simulink model "Oldham_Coupling"  (R2024b)
settings: Solver=ode15s  StartTime=0.0  StopTime=4  MaxStep=0.02  RelTol=1e-3
undefined symbols (not defined in the file or in its folder): X, Y, Z
libraries: sm_lib x14, nesl_utility x2, simulink x1
settings Model: Creator=admin  LastModifiedBy=admin

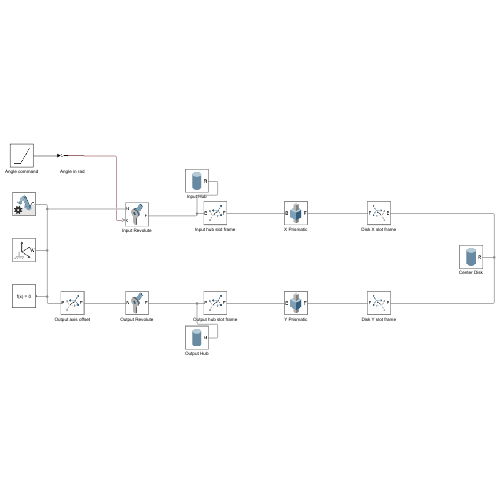
[thumbnail: Simulink's stored preview of the top-level diagram]
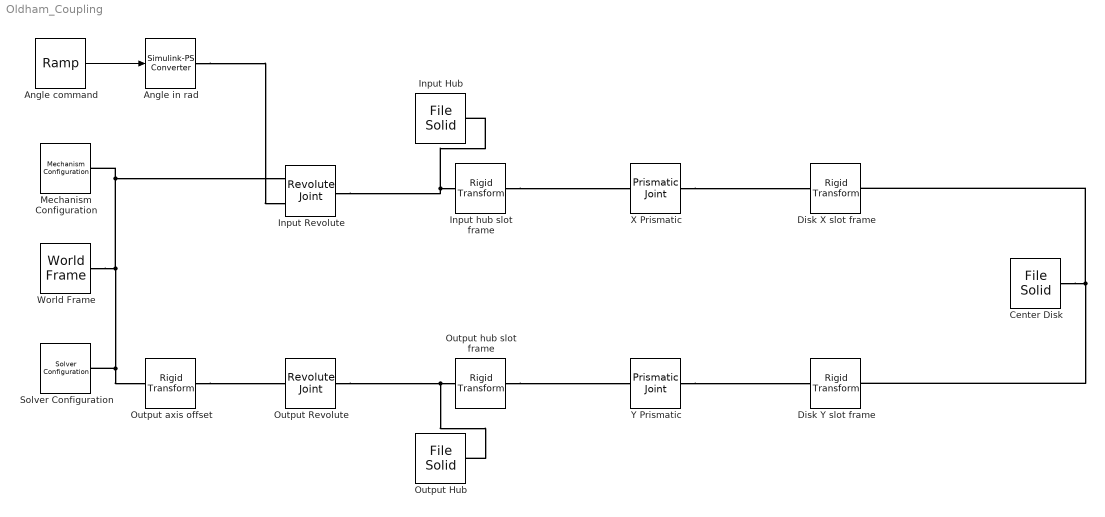
== system Oldham_Coupling ==
  Angle command : simulink/Sources/Ramp  slope=pi  start=0  InitialOutput=0
  Angle in rad : nesl_utility/Simulink-PS Converter  PhysicalDomain=network_engine_domain  SubClassName=ps_input  LeftPortType=input  RightPortType=output  PseudoPeriodic=off  Frequencies=[]  NoiseDistribution=none  NoiseParameters=[]  Unit=rad  AffineConversion=off  FilteringAndDerivatives=filter  SimscapeFilterOrder=2  InputFilterTimeConstant=0.001  UdotUserProvided=0
  Center Disk : sm_lib/Body Elements/File Solid  InertiaType=CalculateFromGeometry  BasedOnType=Density  Density=1000  DensityUnits=kg/m^3  Mass=1  MassUnits=kg  CenterOfMass=[0 0 0]  CenterOfMassUnits=m  MomentsOfInertia=[1 1 1]  MomentsOfInertiaUnits=kg*m^2  ProductsOfInertia=[0 0 0]  ProductsOfInertiaUnits=kg*m^2  GraphicType=FromGeometry  MarkerShape=Sphere  MarkerSize=10  GraphicVisPropType=SimpleVisualProperties  GraphicDiffuseColor=[0.5 0.5 0.5]  GraphicOpacity=1  GraphicSpecularColor=[0.5 0.5 0.5 1.0]  GraphicAmbientColor=[0.15 0.15 0.15 1.0]  GraphicEmissiveColor=[0.0 0.0 0.0 1.0]  GraphicShininess=75  DoExposeReferenceFrame=on  SerializedFrames=<Frames/>  StepReaderType=HEX  ExportConvexHullGeometry=off  ExtGeomFileUnits=mm  ExtGeomFileName=C:\Users\admin\OneDrive\เอกสาร\ChatGPT\Machinery project\cad\Centerdisk.STEP  UnitType=FromFile
  Disk X slot frame : sm_lib/Frames and Transforms/Rigid Transform  RotationMethod=StandardAxis  FollAlignAxisA=+X  BaseAlignAxisA=+Y  FollAlignAxisB=+Y  BaseAlignAxisB=+Z  RotationStandardAxis=+Y  RotationAngle=90  RotationAngleUnits=deg  RotationArbitraryAxis=[0 0 1]  RotationSequenceAxes=FollowerAxes  RotationSequence=XYX  RotationSequenceAngles=[0 0 0]  RotationSequenceAnglesUnits=deg  RotationMatrix=[1 0 0;0 1 0;0 0 1]  Quaternion=[1 0 0 0]  TranslationMethod=Cartesian  TranslationCartesianOffset=[0 0 -6]  TranslationCartesianOffsetUnits=mm  TranslationStandardAxis=+Z  TranslationStandardOffset=0  TranslationStandardOffsetUnits=m  TranslationROffset=0  TranslationROffsetUnits=m  TranslationThetaOffset=0  TranslationThetaOffsetUnits=deg  TranslationZOffset=0  TranslationZOffsetUnits=m
  Disk Y slot frame : sm_lib/Frames and Transforms/Rigid Transform  RotationMethod=StandardAxis  FollAlignAxisA=+X  BaseAlignAxisA=+Y  FollAlignAxisB=+Y  BaseAlignAxisB=+Z  RotationStandardAxis=+X  RotationAngle=-90  RotationAngleUnits=deg  RotationArbitraryAxis=[0 0 1]  RotationSequenceAxes=FollowerAxes  RotationSequence=XYX  RotationSequenceAngles=[0 0 0]  RotationSequenceAnglesUnits=deg  RotationMatrix=[1 0 0;0 1 0;0 0 1]  Quaternion=[1 0 0 0]  TranslationMethod=Cartesian  TranslationCartesianOffset=[0 0 6]  TranslationCartesianOffsetUnits=mm  TranslationStandardAxis=+Z  TranslationStandardOffset=0  TranslationStandardOffsetUnits=m  TranslationROffset=0  TranslationROffsetUnits=m  TranslationThetaOffset=0  TranslationThetaOffsetUnits=deg  TranslationZOffset=0  TranslationZOffsetUnits=m
  Input Hub : sm_lib/Body Elements/File Solid  InertiaType=CalculateFromGeometry  BasedOnType=Density  Density=1000  DensityUnits=kg/m^3  Mass=1  MassUnits=kg  CenterOfMass=[0 0 0]  CenterOfMassUnits=m  MomentsOfInertia=[1 1 1]  MomentsOfInertiaUnits=kg*m^2  ProductsOfInertia=[0 0 0]  ProductsOfInertiaUnits=kg*m^2  GraphicType=FromGeometry  MarkerShape=Sphere  MarkerSize=10  GraphicVisPropType=SimpleVisualProperties  GraphicDiffuseColor=[0.5 0.5 0.5]  GraphicOpacity=1  GraphicSpecularColor=[0.5 0.5 0.5 1.0]  GraphicAmbientColor=[0.15 0.15 0.15 1.0]  GraphicEmissiveColor=[0.0 0.0 0.0 1.0]  GraphicShininess=75  DoExposeReferenceFrame=on  SerializedFrames=<Frames/>  StepReaderType=HEX  ExportConvexHullGeometry=off  ExtGeomFileUnits=mm  ExtGeomFileName=C:\Users\admin\OneDrive\เอกสาร\ChatGPT\Machinery project\cad\Input.STEP  UnitType=FromFile
  Input Revolute : sm_lib/Joints/Revolute Joint  JointMode=Normal  CompositeWrenchDir=FollowerOnBase  CompositeWrenchFrame=BaseFrame  SenseConstraintForce=off  SenseConstraintTorque=off  SenseTotalForce=off  SenseTotalTorque=off  PositionTargetSpecify=off  PositionTargetPriority=High  PositionTargetValue=0  PositionTargetValueUnits=deg  VelocityTargetSpecify=off  VelocityTargetPriority=High  VelocityTargetValue=0  VelocityTargetValueUnits=deg/s  EquilibriumPosition=0  EquilibriumPositionUnits=deg  SpringStiffness=0  SpringStiffnessUnits=N*m/deg  DampingCoefficient=0  DampingCoefficientUnits=N*m/(deg/s)  LowerLimitSpecify=off  LowerLimitBound=-90  LowerLimitBoundUnits=deg  LowerLimitStiffness=1e4  LowerLimitStiffnessUnits=N*m/deg  LowerLimitDamping=10  LowerLimitDampingUnits=N*m/(deg/s)  LowerLimitTransitionRegionWidth=0.1  LowerLimitTransitionRegionWidthUnits=deg  UpperLimitSpecify=off  UpperLimitBound=90  UpperLimitBoundUnits=deg  UpperLimitStiffness=1e4  UpperLimitStiffnessUnits=N*m/deg  UpperLimitDamping=10  UpperLimitDampingUnits=N*m/(deg/s)  UpperLimitTransitionRegionWidth=0.1  UpperLimitTransitionRegionWidthUnits=deg  TorqueActuationMode=ComputedTorque  MotionActuationMode=InputMotion  SensePosition=off  SenseVelocity=off  SenseAcceleration=off  SenseTorqueForce=off  SenseLowerLimitTorqueForce=off  SenseUpperLimitTorqueForce=off
  Input hub slot frame : sm_lib/Frames and Transforms/Rigid Transform  RotationMethod=StandardAxis  FollAlignAxisA=+X  BaseAlignAxisA=+Y  FollAlignAxisB=+Y  BaseAlignAxisB=+Z  RotationStandardAxis=+Y  RotationAngle=90  RotationAngleUnits=deg  RotationArbitraryAxis=[0 0 1]  RotationSequenceAxes=FollowerAxes  RotationSequence=XYX  RotationSequenceAngles=[0 0 0]  RotationSequenceAnglesUnits=deg  RotationMatrix=[1 0 0;0 1 0;0 0 1]  Quaternion=[1 0 0 0]  TranslationMethod=Cartesian  TranslationCartesianOffset=[0 0 5]  TranslationCartesianOffsetUnits=mm  TranslationStandardAxis=+Z  TranslationStandardOffset=0  TranslationStandardOffsetUnits=m  TranslationROffset=0  TranslationROffsetUnits=m  TranslationThetaOffset=0  TranslationThetaOffsetUnits=deg  TranslationZOffset=0  TranslationZOffsetUnits=m
  Mechanism Configuration : sm_lib/Utilities/Mechanism Configuration  UniformGravity=Constant  GravityVector=[0 0 -9.80665]  GravityVectorUnits=m/s^2  LinearizationDelta=0.001  JointModeTransitionNonlinearIterations=2
  Output Hub : sm_lib/Body Elements/File Solid  InertiaType=CalculateFromGeometry  BasedOnType=Density  Density=1000  DensityUnits=kg/m^3  Mass=1  MassUnits=kg  CenterOfMass=[0 0 0]  CenterOfMassUnits=m  MomentsOfInertia=[1 1 1]  MomentsOfInertiaUnits=kg*m^2  ProductsOfInertia=[0 0 0]  ProductsOfInertiaUnits=kg*m^2  GraphicType=FromGeometry  MarkerShape=Sphere  MarkerSize=10  GraphicVisPropType=SimpleVisualProperties  GraphicDiffuseColor=[0.5 0.5 0.5]  GraphicOpacity=1  GraphicSpecularColor=[0.5 0.5 0.5 1.0]  GraphicAmbientColor=[0.15 0.15 0.15 1.0]  GraphicEmissiveColor=[0.0 0.0 0.0 1.0]  GraphicShininess=75  DoExposeReferenceFrame=on  SerializedFrames=<Frames/>  StepReaderType=HEX  ExportConvexHullGeometry=off  ExtGeomFileUnits=mm  ExtGeomFileName=C:\Users\admin\OneDrive\เอกสาร\ChatGPT\Machinery project\cad\Output.STEP  UnitType=FromFile
  Output Revolute : sm_lib/Joints/Revolute Joint  JointMode=Normal  CompositeWrenchDir=FollowerOnBase  CompositeWrenchFrame=BaseFrame  SenseConstraintForce=off  SenseConstraintTorque=off  SenseTotalForce=off  SenseTotalTorque=off  PositionTargetSpecify=off  PositionTargetPriority=High  PositionTargetValue=0  PositionTargetValueUnits=deg  VelocityTargetSpecify=off  VelocityTargetPriority=High  VelocityTargetValue=0  VelocityTargetValueUnits=deg/s  EquilibriumPosition=0  EquilibriumPositionUnits=deg  SpringStiffness=0  SpringStiffnessUnits=N*m/deg  DampingCoefficient=0  DampingCoefficientUnits=N*m/(deg/s)  LowerLimitSpecify=off  LowerLimitBound=-90  LowerLimitBoundUnits=deg  LowerLimitStiffness=1e4  LowerLimitStiffnessUnits=N*m/deg  LowerLimitDamping=10  LowerLimitDampingUnits=N*m/(deg/s)  LowerLimitTransitionRegionWidth=0.1  LowerLimitTransitionRegionWidthUnits=deg  UpperLimitSpecify=off  UpperLimitBound=90  UpperLimitBoundUnits=deg  UpperLimitStiffness=1e4  UpperLimitStiffnessUnits=N*m/deg  UpperLimitDamping=10  UpperLimitDampingUnits=N*m/(deg/s)  UpperLimitTransitionRegionWidth=0.1  UpperLimitTransitionRegionWidthUnits=deg  TorqueActuationMode=NoTorque  MotionActuationMode=ComputedMotion  SensePosition=off  SenseVelocity=off  SenseAcceleration=off  SenseTorqueForce=off  SenseLowerLimitTorqueForce=off  SenseUpperLimitTorqueForce=off
  Output axis offset : sm_lib/Frames and Transforms/Rigid Transform  RotationMethod=None  FollAlignAxisA=+X  BaseAlignAxisA=+Y  FollAlignAxisB=+Y  BaseAlignAxisB=+Z  RotationStandardAxis=+Z  RotationAngle=0  RotationAngleUnits=deg  RotationArbitraryAxis=[0 0 1]  RotationSequenceAxes=FollowerAxes  RotationSequence=XYX  RotationSequenceAngles=[0 0 0]  RotationSequenceAnglesUnits=deg  RotationMatrix=[1 0 0;0 1 0;0 0 1]  Quaternion=[1 0 0 0]  TranslationMethod=Cartesian  TranslationCartesianOffset=[5 0 22]  TranslationCartesianOffsetUnits=mm  TranslationStandardAxis=+Z  TranslationStandardOffset=0  TranslationStandardOffsetUnits=m  TranslationROffset=0  TranslationROffsetUnits=m  TranslationThetaOffset=0  TranslationThetaOffsetUnits=deg  TranslationZOffset=0  TranslationZOffsetUnits=m
  Output hub slot frame : sm_lib/Frames and Transforms/Rigid Transform  RotationMethod=StandardAxis  FollAlignAxisA=+X  BaseAlignAxisA=+Y  FollAlignAxisB=+Y  BaseAlignAxisB=+Z  RotationStandardAxis=+X  RotationAngle=-90  RotationAngleUnits=deg  RotationArbitraryAxis=[0 0 1]  RotationSequenceAxes=FollowerAxes  RotationSequence=XYX  RotationSequenceAngles=[0 0 0]  RotationSequenceAnglesUnits=deg  RotationMatrix=[1 0 0;0 1 0;0 0 1]  Quaternion=[1 0 0 0]  TranslationMethod=Cartesian  TranslationCartesianOffset=[0 0 -5]  TranslationCartesianOffsetUnits=mm  TranslationStandardAxis=+Z  TranslationStandardOffset=0  TranslationStandardOffsetUnits=m  TranslationROffset=0  TranslationROffsetUnits=m  TranslationThetaOffset=0  TranslationThetaOffsetUnits=deg  TranslationZOffset=0  TranslationZOffsetUnits=m
  Solver Configuration : nesl_utility/Solver Configuration  PhysicalDomain=network_engine_domain  SubClassName=solver  LeftPortType=input  RightPortType=generic  Tones=[]  Harmonics=[]  SimulateNoise=off  Profile=off  UseLocalSampling=off  EnableSwitchedLinearOptims=on  FrequencyDomain=off  UseCCode=off  RelTol=0.001  AbsTol=0.001  MinStep=1e-09  ToWorkspace=off  RevertToSquareIcSolve=off  NumHomotopyIterations=100  PhasorMode=off  PhasorModeNumHarmonics=1  ConsistencySolver=NEWTON_XTOL_AFTER_FTOL  IndexReductionMethod=DerivativeReplacement  DoDC=off  ResidualTolerance=1e-09  ConsistencyTolSource=GLOBAL  ConsistencyAbsTol=0.001  ConsistencyRelTol=0.001  ConsistencyTolFactor=0.001  UseLocalSolver=off  LocalSolverChoice=NE_BACKWARD_EULER_ADVANCER  ResolveIndetEquations=on  FunctionEvalNumThread=1  LocalSolverSampleTime=0.001  DoFixedCost=off  MaxNonlinIter=3  MaxModeIter=2  ComputeImpulses=off  ImpulseIterations=2  LinearAlgebra=auto  LinearAlgebraNumThread=0  EquationFormulation=NE_TIME_EF  DelaysMemoryBudget=1024  AutomaticFiltering=on  FilteringTimeConstant=0.001  PartitionStorageMethod=AS_NEEDED  PartitionMemoryBudget=1024  PartitionMethod=ROBUST  MultibodyUseLocalSolver=off  MultibodyLocalSolverChoice=ODE1  MultibodyLocalSolverSampleTime=0.001
  World Frame : sm_lib/Frames and Transforms/World Frame
  X Prismatic : sm_lib/Joints/Prismatic Joint  JointMode=Normal  CompositeWrenchDir=FollowerOnBase  CompositeWrenchFrame=BaseFrame  SenseConstraintForce=off  SenseConstraintTorque=off  SenseTotalForce=off  SenseTotalTorque=off  PositionTargetSpecify=off  PositionTargetPriority=High  PositionTargetValue=0  PositionTargetValueUnits=m  VelocityTargetSpecify=off  VelocityTargetPriority=High  VelocityTargetValue=0  VelocityTargetValueUnits=m/s  EquilibriumPosition=0  EquilibriumPositionUnits=m  SpringStiffness=0  SpringStiffnessUnits=N/m  DampingCoefficient=0  DampingCoefficientUnits=N/(m/s)  LowerLimitSpecify=off  LowerLimitBound=-1  LowerLimitBoundUnits=m  LowerLimitStiffness=1e6  LowerLimitStiffnessUnits=N/m  LowerLimitDamping=1e3  LowerLimitDampingUnits=N/(m/s)  LowerLimitTransitionRegionWidth=1e-4  LowerLimitTransitionRegionWidthUnits=m  UpperLimitSpecify=off  UpperLimitBound=1  UpperLimitBoundUnits=m  UpperLimitStiffness=1e6  UpperLimitStiffnessUnits=N/m  UpperLimitDamping=1e3  UpperLimitDampingUnits=N/(m/s)  UpperLimitTransitionRegionWidth=1e-4  UpperLimitTransitionRegionWidthUnits=m  TorqueActuationMode=NoTorque  MotionActuationMode=ComputedMotion  SensePosition=off  SenseVelocity=off  SenseAcceleration=off  SenseTorqueForce=off  SenseLowerLimitTorqueForce=off  SenseUpperLimitTorqueForce=off
  Y Prismatic : sm_lib/Joints/Prismatic Joint  JointMode=Normal  CompositeWrenchDir=FollowerOnBase  CompositeWrenchFrame=BaseFrame  SenseConstraintForce=off  SenseConstraintTorque=off  SenseTotalForce=off  SenseTotalTorque=off  PositionTargetSpecify=off  PositionTargetPriority=High  PositionTargetValue=0  PositionTargetValueUnits=m  VelocityTargetSpecify=off  VelocityTargetPriority=High  VelocityTargetValue=0  VelocityTargetValueUnits=m/s  EquilibriumPosition=0  EquilibriumPositionUnits=m  SpringStiffness=0  SpringStiffnessUnits=N/m  DampingCoefficient=0  DampingCoefficientUnits=N/(m/s)  LowerLimitSpecify=off  LowerLimitBound=-1  LowerLimitBoundUnits=m  LowerLimitStiffness=1e6  LowerLimitStiffnessUnits=N/m  LowerLimitDamping=1e3  LowerLimitDampingUnits=N/(m/s)  LowerLimitTransitionRegionWidth=1e-4  LowerLimitTransitionRegionWidthUnits=m  UpperLimitSpecify=off  UpperLimitBound=1  UpperLimitBoundUnits=m  UpperLimitStiffness=1e6  UpperLimitStiffnessUnits=N/m  UpperLimitDamping=1e3  UpperLimitDampingUnits=N/(m/s)  UpperLimitTransitionRegionWidth=1e-4  UpperLimitTransitionRegionWidthUnits=m  TorqueActuationMode=NoTorque  MotionActuationMode=ComputedMotion  SensePosition=off  SenseVelocity=off  SenseAcceleration=off  SenseTorqueForce=off  SenseLowerLimitTorqueForce=off  SenseUpperLimitTorqueForce=off
  wires:
  Angle command/1 -> Angle in rad/1
  connections:
  Mechanism Configuration/RConn1 -- World Frame/RConn1 -- Solver Configuration/RConn1 -- Output axis offset/LConn1 -- Input Revolute/LConn1
  Output axis offset/RConn1 -- Output Revolute/LConn1
  Input Hub/RConn1 -- Input Revolute/RConn1 -- Input hub slot frame/LConn1
  Output Hub/RConn1 -- Output Revolute/RConn1 -- Output hub slot frame/LConn1
  Input hub slot frame/RConn1 -- X Prismatic/LConn1
  Output hub slot frame/RConn1 -- Y Prismatic/LConn1
  X Prismatic/RConn1 -- Disk X slot frame/RConn1
  Y Prismatic/RConn1 -- Disk Y slot frame/RConn1
  Disk X slot frame/LConn1 -- Center Disk/RConn1 -- Disk Y slot frame/LConn1
  Angle in rad/RConn1 -- Input Revolute/LConn2
